simulink model "DualActiveBridgeConverter"  (R2026a)
settings: Solver=ode23t  StopTime=0.010  MaxStep=1e-5  AbsTol=1e-3
PreLoadFcn:
  | DABDefaultInputParameters;
model workspace (MAT data in the model file):
  ConverterKey : string (value not decoded)
undefined symbols (not defined in the file): DABController, DABDesign
libraries: ee_lib x45, nesl_utility x38, fl_lib x19, ConverterLibrary x1, simulink_extras x1
(part 3 of 5)

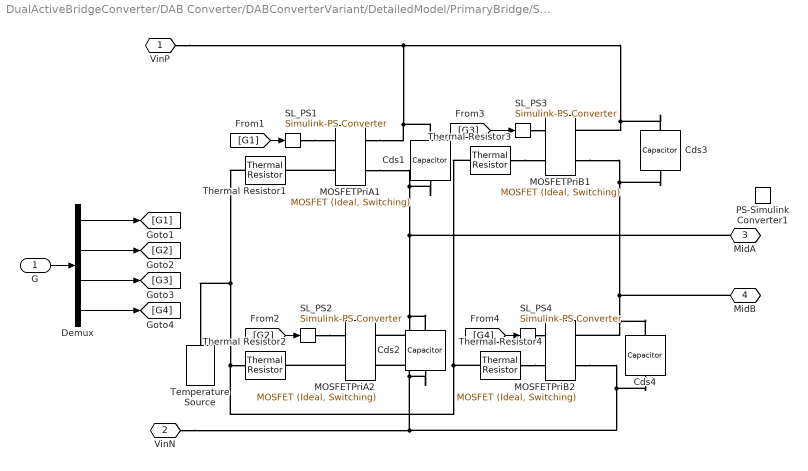
== system DualActiveBridgeConverter/DAB Converter/DABConverterVariant/DetailedModel/PrimaryBridge/SwitchingMOSFETwithThermal ==
  G : Inport
  Cds{1..4} (4 alike) : ee_lib/Passive/Capacitor  cap_option=ee.enum.passive.capacitor.capOption.const  c=CossPri_SI F  Cvec=[1e-05, 1e-06] F  Vvec=[0, 10] V  CV_table_symmetry=ee.enum.passive.capacitor.tableSymmetry.yes  f_vec=[1, 10] kHz  DFext_vec=[.8, 1.2]  enable_C_tol=ee.enum.toleranceApplication.none  averaging_period=0 s  C_tol=5  tol_distribution=ee.enum.toleranceDistribution.uniform  nSigma=4  r=0.05 Ohm  g=1e-5 1/Ohm  enable_operating_limits=ee.enum.enable.no  operating_limit_action=ee.enum.passive.reportOpLim.warn  max_working_voltage_range=[-25, 25] V  power_rating=1 W  maxTemperature=85 degC  thermalEnable=false  thermalMass=1 J/K  i_specify=off  i_priority=None  i=0 A  i_nominal_specify=off  i_nominal_value=1  i_nominal_unit=A  v_specify=off  v_priority=None  v=0 V  v_nominal_specify=off  v_nominal_value=1  v_nominal_unit=V  vc_specify=on  vc_priority=None  vc=0 V  vc_nominal_specify=off  vc_nominal_value=1  vc_nominal_unit=V  T_specify=off  T_priority=None  T=298.15 K  T_nominal_specify=off  T_nominal_value=1  T_nominal_unit=K
  Demux : Demux
  MOSFETPriA1 : ee_lib/Semiconductors & Converters/MOSFET (Ideal, Switching)  PartSpecification="{\"CollectionId\":\"MW.SimscapeElectrical\",\"CollectionVersion\":\"1.0.0\",\"DatasetId\":\"Wolfspeed|C2M0080120D|simscape.electrical.mosfetIdealSwitching\",\"DisplayName\":\"Wolfspeed:C2M0080120D\"}"  port_option=ee.enum.controlport.ps  Rds=0.08 % Datasheet derived Ohm  Goff=8.33333333333333e-10 % Datasheet derived S  Vth=2.9 % Datasheet derived V  diode_param=ee.enum.semiconductors.protectionDiode.nodynamics  diode_Vf=2.47 % Datasheet derived V  diode_Ron=0.031 % Wolfspeed XML derived Ohm  diode_Goff=1e-05 % Library default S  diode_C=50e-9 % Parameter not set F  diode_iRM=-235 % Parameter not set A  diode_iF=300 % Parameter not set A  diode_idot=-50 % Parameter not set A/us  diode_trr_param=ee.enum.converters.diodeReverseParam.trr_factor  diode_trr_factor=3 % Parameter not set  diode_trr=15 % Parameter not set us  diode_Qrr=1500 % Parameter not set s*uA  ids_specify=off  ids_priority=None  ids=0 A  ids_nominal_specify=off  ids_nominal_value=1  ids_nominal_unit=A  vds_specify=off  vds_priority=None  vds=0 V  vds_nominal_specify=off  vds_nominal_value=1  vds_nominal_unit=V  vgs_specify=off  vgs_priority=None  vgs=0 V  vgs_nominal_specify=off  vgs_nominal_value=1  vgs_nominal_unit=V  thermal_loss_option=ee.enum.converters.thermalLossOption.tabulated2d  Von_data=[-3.8 -2.8 -1.8 -1.25 -0.68 -0.35 -0.215 -0.07 0 0.05406 0.21 0.38 0.78 1.6 2.42 3.47 4.66 4.96;-5 -3.49 -2.12 -1.43 -0.746 -0.376 -0.225 -0.074 0 0.075 0.153 0.386 0.785 1.66 2.65 3.85 5.34 5.7;-5.3 -4.56 -3.66 -2.61 -1.344 -0.68 -0.41 -0.15 0 0.152 0.31 0.74 1.44 3 4.97 7.58 11.32 12.44;-6.36 -5.472 -4.392 -3.132 -1.6128 -0.816 -0.492 -0.18 0 0.1824 0.372 0.888 1.728 3.6 5.964 9.096 13.584 14.928] % Wolfspeed XML derived V  Tj=[-55 25 150 900] % Wolfspeed XML derived degC  Iout_data=[-70 -50 -30 -20 -10 -5 -3 -1 0 1 3 5 10 20 30 40 50 52] % Wolfspeed XML derived A  tabulateWithVds=true  Eon_data=[0 0.000124976993 0.00019839481 0.000290262596 0.000394695025 0.000523309904 0.000664552409 0.000828222079 0.001003319539;0 0.000124640962 0.0001962155 0.000286135235 0.000385392686 0.000510053121 0.00064771759 0.000807241087 0.000977902879;0 0.000123102531 0.000190031631 0.000279362347 0.000372104061 0.000492143088 0.0006249736 0.000778895581 0.000943564745;0 0.000122189781 0.000189721879 0.000280387095 0.000371182205 0.000491705578 0.000624418005 0.00077820315 0.000942725925;0 9.7751825e-05 0.000151777503 0.000224309676 0.000296945764 0.000393364462 0.000499534404 0.00062256252 0.00075418074] % Wolfspeed XML derived J  Eoff_data=[0 2.7034922e-05 2.6405907e-05 2.8222037e-05 4.6178646e-05 7.2338984e-05 0.000103764515 0.000172183844 0.000226354181;0 2.7736404e-05 2.7071047e-05 2.901408e-05 4.8053099e-05 7.444232e-05 0.000106781584 0.000177190281 0.000232935681;0 2.8327181e-05 2.7741775e-05 2.9983555e-05 5.0035781e-05 7.7828104e-05 0.000111638221 0.000185249245 0.000243530056;0 2.8334748e-05 2.8341663e-05 3.154355e-05 5.2631616e-05 8.0707822e-05 0.000115768947 0.000192103652 0.000252540911;0 3.4001697e-05 3.4009995e-05 3.785226e-05 6.3157939e-05 9.6849386e-05 0.000138922737 0.000230524383 0.000303049093] % Wolfspeed XML derived J  Eon_data_3D=reshape([0;0;0;0;0;0;0;0;0;0;0;0;0;0;0;0;0;0;0;0;0;0;0;0;0;0;0;0;0;0;0;0;0;0;0;0;0;0;0;0;0;0;0;0;0;0;0;0;0;0;0;0;0;0;0;0;0;0;0;0;0;0;0;0;0;0;0;0;0;0;0;0;0;0;0;0;0;0;0;0;0;0;0;0;0;0;0;0;0;0;0;0;0;0;0;8.0560812e-05;8.0344205e-05;7.9352525e-05;7.8764161e-05;6.3011329e-05;0.00013000148;0.000128573451;0.000124521369;0.000124318399;9.9454719e-05;0.000196389357;0.000193596818;0.000189014336;0.000189707672;0.000151766137;0.000270014001;0.000263650198;0.000254559344;0.000253928694;0.000203142956;0.000365443107;0.000356185495;0.000343678379;0.000343372852;0.000274698281;0.000469433942;0.000457541975;0.000441475822;0.000441083354;0.000352866683;0.00058790882;0.00057301558;0.000552894681;0.000552403162;0.00044192253;0.000724469353;0.000706116684;0.000681322066;0.000680716377;0.000544573101;0;0;0;0;0;0.000124976993;0.000124640962;0.000123102531;0.000122189781;9.7751825e-05;0.00019839481;0.0001962155;0.000190031631;0.000189721879;0.000151777503;0.000290262596;0.000286135235;0.000279362347;0.000280387095;0.000224309676;0.000394695025;0.000385392686;0.000372104061;0.000371182205;0.000296945764;0.000523309904;0.000510053121;0.000492143088;0.000491705578;0.000393364462;0.000664552409;0.00064771759;0.0006249736;0.000624418005;0.000499534404;0.000828222079;0.000807241087;0.000778895581;0.00077820315;0.00062256252;0.001003319539;0.000977902879;0.000943564745;0.000942725925;0.00075418074],[5 9 4]) % Wolfspeed XML derived J  Eoff_data_3D=reshape([0;0;0;0;0;0;0;0;0;0;0;0;0;0;0;0;0;0;0;0;0;0;0;0;0;0;0;0;0;0;0;0;0;0;0;0;0;0;0;0;0;0;0;0;0;0;0;0;0;0;0;0;0;0;0;0;0;0;0;0;0;0;0;0;0;0;0;0;0;0;0;0;0;0;0;0;0;0;0;0;0;0;0;0;0;0;0;0;0;0;0;0;0;0;0;1.7265625e-05;1.7713621e-05;1.8090916e-05;1.8095748e-05;2.1714898e-05;1.5629082e-05;1.6022764e-05;1.6419753e-05;1.6774814e-05;2.0129777e-05;1.8332459e-05;1.8846954e-05;1.9476705e-05;2.0490046e-05;2.4588055e-05;3.1702259e-05;3.2989096e-05;3.4350234e-05;3.6132309e-05;4.3358771e-05;5.1589831e-05;5.3089863e-05;5.5504495e-05;5.7558217e-05;6.906986e-05;8.8425554e-05;9.0996626e-05;9.5135332e-05;9.8655434e-05;0.000118386521;0.000127762888;0.000131477737;0.000137457604;0.000142543673;0.000171052407;0.000173370104;0.000178411033;0.000186525519;0.00019342715;0.000232112579;0;0;0;0;0;2.7034922e-05;2.7736404e-05;2.8327181e-05;2.8334748e-05;3.4001697e-05;2.6405907e-05;2.7071047e-05;2.7741775e-05;2.8341663e-05;3.4009995e-05;2.8222037e-05;2.901408e-05;2.9983555e-05;3.154355e-05;3.785226e-05;4.6178646e-05;4.8053099e-05;5.0035781e-05;5.2631616e-05;6.3157939e-05;7.2338984e-05;7.444232e-05;7.7828104e-05;8.0707822e-05;9.6849386e-05;0.000103764515;0.000106781584;0.000111638221;0.000115768947;0.000138922737;0.000172183844;0.000177190281;0.000185249245;0.000192103652;0.000230524383;0.000226354181;0.000232935681;0.000243530056;0.000252540911;0.000303049093],[5 9 4]) % Wolfspeed XML derived J  Tj_loss=[25 75 125 150 900] % Wolfspeed XML derived degC  Iout_data_loss=[0 4.08 8.4 12.48 16.32 20.4 24.24 27.84 31.68] % Wolfspeed XML derived A  Vds_loss=[-10 0 600 800] % Wolfspeed XML derived V  Eon_scalar=22.86e-3 % Parameter not set J  Eoff_scalar=17.14e-3 % Parameter not set J  Voff=300 % Parameter not set V  Iout_scalar=600 % Parameter not set A  useCurrentFromPreviousCycle=false  useVoltageFromPreviousCycle=false  diodeModelType=ee.enum.converters.diodeModelType.tabulated  diodeTableType=ee.enum.diode.tableType.VfMat  diode_ReverseIVType=ee.enum.diode.diodeReverseIV.constant  diode_IfMat=[.07, .12, .19, 1.75, 4.24, 7.32, 11.2; .16, .3, .72, 2.14, 4.02, 6.35, 9.12] % Parameter not set A  diode_VfMat=[0 3.27 3.6 3.85 4.4 4.95 5.7 6.25 7 7.62;0 2.8 3.16 3.4 3.8 4.25 4.85 5.3 6 6.6;0 2.52 2.76 2.97 3.36 3.78 4.35 4.8 5.5 6.1;0 2.016 2.208 2.376 2.688 3.024 3.48 3.84 4.4 4.88] % Wolfspeed XML derived V  diode_TjVec=[-55 25 150 900] % Wolfspeed XML derived degC  diode_VfVec=[.5, .7, .9, 1.3, 1.7, 2.1, 2.5] % Parameter not set V  diode_IfVec=[0 0.3 1 2 5 10 20 30 50 70] % Wolfspeed XML derived A  diode_IrMat=[1e-06, 2e-06, 5e-06, 1e-05, 2.5e-05, 5e-05, .0001; 2e-06, 5e-06, 1e-05, 4e-05, 8e-05, .0002, .0005] % Parameter not set A  diode_VrMat=[10, 100, 200, 250, 300, 325, 350; 10, 70, 160, 220, 270, 300, 320] % Parameter not set V  diode_VrVec=[10, 20, 40, 50, 70, 80, 100] % Parameter not set V  diode_IrVec=[1e-06, 2e-06, 5e-06, 1e-05, 2e-05, 5e-05, .0001] % Parameter not set A  diode_Vr=-600 % Parameter not set V  diode_Ls=150 % Parameter not set nH  diode_Erec=0.03 % Parameter not set J  diode_rec_loss_model=ee.enum.diode.reverseRecoveryModelTabulateUpTo3D.fixed  diode_ErecVal=0 % Parameter not set J  diode_scaleWithIandV=false  diode_ErecMat=[0 0;0 0] % Wolfspeed XML derived J  diodeErecMat3D=zeros(2, 3, 2) % Parameter not set J  diode_TjrecVec=[25 35] % Wolfspeed XML derived degC  diode_IfrecVec=[0 10] % Wolfspeed XML derived A  diodeVrecVec=[0, 100] % Parameter not set V  diode_IrecVal=10 % Parameter not set A  diode_VrecVal=10 % Wolfspeed XML derived V  diode_tFilter=1 / 1000 / 100 % Parameter not set s  separateThermalPortForDiode=false  thermal_network_parameterization=ee.enum.thermalNetworkTopology.external  Rth=[.03, .2] % Parameter not set K/W  Rth_Cauer=[0.00956 0.242 0.167 0.228] % Wolfspeed XML derived K/W  Rth_Foster=[.08, .14, .22, .16] % Parameter not set K/W  thermal_mass_parameterization=ee.enum.thermalNetwork.thermalmass  thermal_mass=[3, 25] % Parameter not set J/K  thermal_mass_Cauer=[0.00156 0.00604 0.0619 0.358] % Wolfspeed XML derived J/K  thermal_mass_Foster=[.001, .005, .05, .5] % Parameter not set J/K  thermal_time_constant=[.1, 5] % Parameter not set s  thermal_time_constant_Cauer=[.1, 1, 5] % Parameter not set s  thermal_time_constant_Foster=[7e-05, .0007, .01, .08] % Parameter not set s  thermal_mass_initial_temperatures=[25, 25] % Parameter not set degC  thermal_mass_initial_temperatures_Cauer=[25 25 25 25] % Wolfspeed XML derived degC  junction_thermal_mass=0.1 % Parameter not set J/K  Tvec_initial_Foster=[25, 25, 25, 25] % Parameter not set degC  RthDiode=[.03, .2] % Parameter not set K/W  RthCauerDiode=[0.00956 0.242 0.167 0.228] % Wolfspeed XML derived K/W  RthFosterDiode=[.03, .2] % Parameter not set K/W  thermalMassDiode=[3, 25] % Parameter not set J/K  thermalMassCauerDiode=[0.00156 0.00604 0.0619 0.358] % Wolfspeed XML derived J/K  thermalMassFosterDiode=[33, 50] % Parameter not set J/K  thermalTauDiode=[.1, 5] % Parameter not set s  thermalTauCauerDiode=[.1, 1, 5] % Parameter not set s  thermalTauFosterDiode=[1, 10] % Parameter not set s  thermalMassInitTempDiode=[25, 25] % Parameter not set degC  thermalMassInitTempCauerDiode=[25 25 25 25] % Wolfspeed XML derived degC  junctionthermalMassDiode=0.1 % Parameter not set J/K  TVecInitialFosterDiode=[25, 25, 25, 25] % Parameter not set degC  no_thermal_network=0 % Parameter not set  mosfet_junction_temperature_specify=on  mosfet_junction_temperature_priority=High  mosfet_junction_temperature=simTempPri_K K  mosfet_junction_temperature_nominal_specify=off  mosfet_junction_temperature_nominal_value=1  mosfet_junction_temperature_nominal_unit=degC  diode_junction_temperature_specify=off  diode_junction_temperature_priority=None  diode_junction_temperature=simTempPri_K K  diode_junction_temperature_nominal_specify=off  diode_junction_temperature_nominal_value=1  diode_junction_temperature_nominal_unit=degC  Qj_specify=off  Qj_priority=None  Qj=0 W  Qj_nominal_specify=off  Qj_nominal_value=1  Qj_nominal_unit=W  accumulatedSwitchingLosses_specify=off  accumulatedSwitchingLosses_priority=None  accumulatedSwitchingLosses=0 J
      settings: AttributesFormatString=Wolfspeed:C2M0080120D
  MOSFETPriA2 : ee_lib/Semiconductors & Converters/MOSFET (Ideal, Switching)  PartSpecification="{\"CollectionId\":\"MW.SimscapeElectrical\",\"CollectionVersion\":\"1.0.0\",\"DatasetId\":\"Wolfspeed|C2M0080120D|simscape.electrical.mosfetIdealSwitching\",\"DisplayName\":\"Wolfspeed:C2M0080120D\"}"  port_option=ee.enum.controlport.ps  Rds=0.08 % Datasheet derived Ohm  Goff=8.33333333333333e-10 % Datasheet derived S  Vth=2.9 % Datasheet derived V  diode_param=ee.enum.semiconductors.protectionDiode.nodynamics  diode_Vf=2.47 % Datasheet derived V  diode_Ron=0.031 % Wolfspeed XML derived Ohm  diode_Goff=1e-05 % Library default S  diode_C=50e-9 % Parameter not set F  diode_iRM=-235 % Parameter not set A  diode_iF=300 % Parameter not set A  diode_idot=-50 % Parameter not set A/us  diode_trr_param=ee.enum.converters.diodeReverseParam.trr_factor  diode_trr_factor=3 % Parameter not set  diode_trr=15 % Parameter not set us  diode_Qrr=1500 % Parameter not set s*uA  ids_specify=off  ids_priority=None  ids=0 A  ids_nominal_specify=off  ids_nominal_value=1  ids_nominal_unit=A  vds_specify=off  vds_priority=None  vds=0 V  vds_nominal_specify=off  vds_nominal_value=1  vds_nominal_unit=V  vgs_specify=off  vgs_priority=None  vgs=0 V  vgs_nominal_specify=off  vgs_nominal_value=1  vgs_nominal_unit=V  thermal_loss_option=ee.enum.converters.thermalLossOption.tabulated2d  Von_data=[-3.8 -2.8 -1.8 -1.25 -0.68 -0.35 -0.215 -0.07 0 0.05406 0.21 0.38 0.78 1.6 2.42 3.47 4.66 4.96;-5 -3.49 -2.12 -1.43 -0.746 -0.376 -0.225 -0.074 0 0.075 0.153 0.386 0.785 1.66 2.65 3.85 5.34 5.7;-5.3 -4.56 -3.66 -2.61 -1.344 -0.68 -0.41 -0.15 0 0.152 0.31 0.74 1.44 3 4.97 7.58 11.32 12.44;-6.36 -5.472 -4.392 -3.132 -1.6128 -0.816 -0.492 -0.18 0 0.1824 0.372 0.888 1.728 3.6 5.964 9.096 13.584 14.928] % Wolfspeed XML derived V  Tj=[-55 25 150 900] % Wolfspeed XML derived degC  Iout_data=[-70 -50 -30 -20 -10 -5 -3 -1 0 1 3 5 10 20 30 40 50 52] % Wolfspeed XML derived A  tabulateWithVds=true  Eon_data=[0 0.000124976993 0.00019839481 0.000290262596 0.000394695025 0.000523309904 0.000664552409 0.000828222079 0.001003319539;0 0.000124640962 0.0001962155 0.000286135235 0.000385392686 0.000510053121 0.00064771759 0.000807241087 0.000977902879;0 0.000123102531 0.000190031631 0.000279362347 0.000372104061 0.000492143088 0.0006249736 0.000778895581 0.000943564745;0 0.000122189781 0.000189721879 0.000280387095 0.000371182205 0.000491705578 0.000624418005 0.00077820315 0.000942725925;0 9.7751825e-05 0.000151777503 0.000224309676 0.000296945764 0.000393364462 0.000499534404 0.00062256252 0.00075418074] % Wolfspeed XML derived J  Eoff_data=[0 2.7034922e-05 2.6405907e-05 2.8222037e-05 4.6178646e-05 7.2338984e-05 0.000103764515 0.000172183844 0.000226354181;0 2.7736404e-05 2.7071047e-05 2.901408e-05 4.8053099e-05 7.444232e-05 0.000106781584 0.000177190281 0.000232935681;0 2.8327181e-05 2.7741775e-05 2.9983555e-05 5.0035781e-05 7.7828104e-05 0.000111638221 0.000185249245 0.000243530056;0 2.8334748e-05 2.8341663e-05 3.154355e-05 5.2631616e-05 8.0707822e-05 0.000115768947 0.000192103652 0.000252540911;0 3.4001697e-05 3.4009995e-05 3.785226e-05 6.3157939e-05 9.6849386e-05 0.000138922737 0.000230524383 0.000303049093] % Wolfspeed XML derived J  Eon_data_3D=reshape([0;0;0;0;0;0;0;0;0;0;0;0;0;0;0;0;0;0;0;0;0;0;0;0;0;0;0;0;0;0;0;0;0;0;0;0;0;0;0;0;0;0;0;0;0;0;0;0;0;0;0;0;0;0;0;0;0;0;0;0;0;0;0;0;0;0;0;0;0;0;0;0;0;0;0;0;0;0;0;0;0;0;0;0;0;0;0;0;0;0;0;0;0;0;0;8.0560812e-05;8.0344205e-05;7.9352525e-05;7.8764161e-05;6.3011329e-05;0.00013000148;0.000128573451;0.000124521369;0.000124318399;9.9454719e-05;0.000196389357;0.000193596818;0.000189014336;0.000189707672;0.000151766137;0.000270014001;0.000263650198;0.000254559344;0.000253928694;0.000203142956;0.000365443107;0.000356185495;0.000343678379;0.000343372852;0.000274698281;0.000469433942;0.000457541975;0.000441475822;0.000441083354;0.000352866683;0.00058790882;0.00057301558;0.000552894681;0.000552403162;0.00044192253;0.000724469353;0.000706116684;0.000681322066;0.000680716377;0.000544573101;0;0;0;0;0;0.000124976993;0.000124640962;0.000123102531;0.000122189781;9.7751825e-05;0.00019839481;0.0001962155;0.000190031631;0.000189721879;0.000151777503;0.000290262596;0.000286135235;0.000279362347;0.000280387095;0.000224309676;0.000394695025;0.000385392686;0.000372104061;0.000371182205;0.000296945764;0.000523309904;0.000510053121;0.000492143088;0.000491705578;0.000393364462;0.000664552409;0.00064771759;0.0006249736;0.000624418005;0.000499534404;0.000828222079;0.000807241087;0.000778895581;0.00077820315;0.00062256252;0.001003319539;0.000977902879;0.000943564745;0.000942725925;0.00075418074],[5 9 4]) % Wolfspeed XML derived J  Eoff_data_3D=reshape([0;0;0;0;0;0;0;0;0;0;0;0;0;0;0;0;0;0;0;0;0;0;0;0;0;0;0;0;0;0;0;0;0;0;0;0;0;0;0;0;0;0;0;0;0;0;0;0;0;0;0;0;0;0;0;0;0;0;0;0;0;0;0;0;0;0;0;0;0;0;0;0;0;0;0;0;0;0;0;0;0;0;0;0;0;0;0;0;0;0;0;0;0;0;0;1.7265625e-05;1.7713621e-05;1.8090916e-05;1.8095748e-05;2.1714898e-05;1.5629082e-05;1.6022764e-05;1.6419753e-05;1.6774814e-05;2.0129777e-05;1.8332459e-05;1.8846954e-05;1.9476705e-05;2.0490046e-05;2.4588055e-05;3.1702259e-05;3.2989096e-05;3.4350234e-05;3.6132309e-05;4.3358771e-05;5.1589831e-05;5.3089863e-05;5.5504495e-05;5.7558217e-05;6.906986e-05;8.8425554e-05;9.0996626e-05;9.5135332e-05;9.8655434e-05;0.000118386521;0.000127762888;0.000131477737;0.000137457604;0.000142543673;0.000171052407;0.000173370104;0.000178411033;0.000186525519;0.00019342715;0.000232112579;0;0;0;0;0;2.7034922e-05;2.7736404e-05;2.8327181e-05;2.8334748e-05;3.4001697e-05;2.6405907e-05;2.7071047e-05;2.7741775e-05;2.8341663e-05;3.4009995e-05;2.8222037e-05;2.901408e-05;2.9983555e-05;3.154355e-05;3.785226e-05;4.6178646e-05;4.8053099e-05;5.0035781e-05;5.2631616e-05;6.3157939e-05;7.2338984e-05;7.444232e-05;7.7828104e-05;8.0707822e-05;9.6849386e-05;0.000103764515;0.000106781584;0.000111638221;0.000115768947;0.000138922737;0.000172183844;0.000177190281;0.000185249245;0.000192103652;0.000230524383;0.000226354181;0.000232935681;0.000243530056;0.000252540911;0.000303049093],[5 9 4]) % Wolfspeed XML derived J  Tj_loss=[25 75 125 150 900] % Wolfspeed XML derived degC  Iout_data_loss=[0 4.08 8.4 12.48 16.32 20.4 24.24 27.84 31.68] % Wolfspeed XML derived A  Vds_loss=[-10 0 600 800] % Wolfspeed XML derived V  Eon_scalar=22.86e-3 % Parameter not set J  Eoff_scalar=17.14e-3 % Parameter not set J  Voff=300 % Parameter not set V  Iout_scalar=600 % Parameter not set A  useCurrentFromPreviousCycle=false  useVoltageFromPreviousCycle=false  diodeModelType=ee.enum.converters.diodeModelType.tabulated  diodeTableType=ee.enum.diode.tableType.VfMat  diode_ReverseIVType=ee.enum.diode.diodeReverseIV.constant  diode_IfMat=[.07, .12, .19, 1.75, 4.24, 7.32, 11.2; .16, .3, .72, 2.14, 4.02, 6.35, 9.12] % Parameter not set A  diode_VfMat=[0 3.27 3.6 3.85 4.4 4.95 5.7 6.25 7 7.62;0 2.8 3.16 3.4 3.8 4.25 4.85 5.3 6 6.6;0 2.52 2.76 2.97 3.36 3.78 4.35 4.8 5.5 6.1;0 2.016 2.208 2.376 2.688 3.024 3.48 3.84 4.4 4.88] % Wolfspeed XML derived V  diode_TjVec=[-55 25 150 900] % Wolfspeed XML derived degC  diode_VfVec=[.5, .7, .9, 1.3, 1.7, 2.1, 2.5] % Parameter not set V  diode_IfVec=[0 0.3 1 2 5 10 20 30 50 70] % Wolfspeed XML derived A  diode_IrMat=[1e-06, 2e-06, 5e-06, 1e-05, 2.5e-05, 5e-05, .0001; 2e-06, 5e-06, 1e-05, 4e-05, 8e-05, .0002, .0005] % Parameter not set A  diode_VrMat=[10, 100, 200, 250, 300, 325, 350; 10, 70, 160, 220, 270, 300, 320] % Parameter not set V  diode_VrVec=[10, 20, 40, 50, 70, 80, 100] % Parameter not set V  diode_IrVec=[1e-06, 2e-06, 5e-06, 1e-05, 2e-05, 5e-05, .0001] % Parameter not set A  diode_Vr=-600 % Parameter not set V  diode_Ls=150 % Parameter not set nH  diode_Erec=0.03 % Parameter not set J  diode_rec_loss_model=ee.enum.diode.reverseRecoveryModelTabulateUpTo3D.fixed  diode_ErecVal=0 % Parameter not set J  diode_scaleWithIandV=false  diode_ErecMat=[0 0;0 0] % Wolfspeed XML derived J  diodeErecMat3D=zeros(2, 3, 2) % Parameter not set J  diode_TjrecVec=[25 35] % Wolfspeed XML derived degC  diode_IfrecVec=[0 10] % Wolfspeed XML derived A  diodeVrecVec=[0, 100] % Parameter not set V  diode_IrecVal=10 % Parameter not set A  diode_VrecVal=10 % Wolfspeed XML derived V  diode_tFilter=1 / 1000 / 100 % Parameter not set s  separateThermalPortForDiode=false  thermal_network_parameterization=ee.enum.thermalNetworkTopology.external  Rth=[.03, .2] % Parameter not set K/W  Rth_Cauer=[0.00956 0.242 0.167 0.228] % Wolfspeed XML derived K/W  Rth_Foster=[.08, .14, .22, .16] % Parameter not set K/W  thermal_mass_parameterization=ee.enum.thermalNetwork.thermalmass  thermal_mass=[3, 25] % Parameter not set J/K  thermal_mass_Cauer=[0.00156 0.00604 0.0619 0.358] % Wolfspeed XML derived J/K  thermal_mass_Foster=[.001, .005, .05, .5] % Parameter not set J/K  thermal_time_constant=[.1, 5] % Parameter not set s  thermal_time_constant_Cauer=[.1, 1, 5] % Parameter not set s  thermal_time_constant_Foster=[7e-05, .0007, .01, .08] % Parameter not set s  thermal_mass_initial_temperatures=[25, 25] % Parameter not set degC  thermal_mass_initial_temperatures_Cauer=[25 25 25 25] % Wolfspeed XML derived degC  junction_thermal_mass=0.1 % Parameter not set J/K  Tvec_initial_Foster=[25, 25, 25, 25] % Parameter not set degC  RthDiode=[.03, .2] % Parameter not set K/W  RthCauerDiode=[0.00956 0.242 0.167 0.228] % Wolfspeed XML derived K/W  RthFosterDiode=[.03, .2] % Parameter not set K/W  thermalMassDiode=[3, 25] % Parameter not set J/K  thermalMassCauerDiode=[0.00156 0.00604 0.0619 0.358] % Wolfspeed XML derived J/K  thermalMassFosterDiode=[33, 50] % Parameter not set J/K  thermalTauDiode=[.1, 5] % Parameter not set s  thermalTauCauerDiode=[.1, 1, 5] % Parameter not set s  thermalTauFosterDiode=[1, 10] % Parameter not set s  thermalMassInitTempDiode=[25, 25] % Parameter not set degC  thermalMassInitTempCauerDiode=[25 25 25 25] % Wolfspeed XML derived degC  junctionthermalMassDiode=0.1 % Parameter not set J/K  TVecInitialFosterDiode=[25, 25, 25, 25] % Parameter not set degC  no_thermal_network=0 % Parameter not set  mosfet_junction_temperature_specify=on  mosfet_junction_temperature_priority=High  mosfet_junction_temperature=simTempPri_K K  mosfet_junction_temperature_nominal_specify=off  mosfet_junction_temperature_nominal_value=1  mosfet_junction_temperature_nominal_unit=degC  diode_junction_temperature_specify=off  diode_junction_temperature_priority=None  diode_junction_temperature=simTempPri_K K  diode_junction_temperature_nominal_specify=off  diode_junction_temperature_nominal_value=1  diode_junction_temperature_nominal_unit=degC  Qj_specify=off  Qj_priority=None  Qj=0 W  Qj_nominal_specify=off  Qj_nominal_value=1  Qj_nominal_unit=W  accumulatedSwitchingLosses_specify=off  accumulatedSwitchingLosses_priority=None  accumulatedSwitchingLosses=0 J
      settings: AttributesFormatString=Wolfspeed:C2M0080120D
  MOSFETPriB1 : ee_lib/Semiconductors & Converters/MOSFET (Ideal, Switching)  PartSpecification="{\"CollectionId\":\"MW.SimscapeElectrical\",\"CollectionVersion\":\"1.0.0\",\"DatasetId\":\"Wolfspeed|C2M0080120D|simscape.electrical.mosfetIdealSwitching\",\"DisplayName\":\"Wolfspeed:C2M0080120D\"}"  port_option=ee.enum.controlport.ps  Rds=0.08 % Datasheet derived Ohm  Goff=8.33333333333333e-10 % Datasheet derived S  Vth=2.9 % Datasheet derived V  diode_param=ee.enum.semiconductors.protectionDiode.nodynamics  diode_Vf=2.47 % Datasheet derived V  diode_Ron=0.031 % Wolfspeed XML derived Ohm  diode_Goff=1e-05 % Library default S  diode_C=50e-9 % Parameter not set F  diode_iRM=-235 % Parameter not set A  diode_iF=300 % Parameter not set A  diode_idot=-50 % Parameter not set A/us  diode_trr_param=ee.enum.converters.diodeReverseParam.trr_factor  diode_trr_factor=3 % Parameter not set  diode_trr=15 % Parameter not set us  diode_Qrr=1500 % Parameter not set s*uA  ids_specify=off  ids_priority=None  ids=0 A  ids_nominal_specify=off  ids_nominal_value=1  ids_nominal_unit=A  vds_specify=off  vds_priority=None  vds=0 V  vds_nominal_specify=off  vds_nominal_value=1  vds_nominal_unit=V  vgs_specify=off  vgs_priority=None  vgs=0 V  vgs_nominal_specify=off  vgs_nominal_value=1  vgs_nominal_unit=V  thermal_loss_option=ee.enum.converters.thermalLossOption.tabulated2d  Von_data=[-3.8 -2.8 -1.8 -1.25 -0.68 -0.35 -0.215 -0.07 0 0.05406 0.21 0.38 0.78 1.6 2.42 3.47 4.66 4.96;-5 -3.49 -2.12 -1.43 -0.746 -0.376 -0.225 -0.074 0 0.075 0.153 0.386 0.785 1.66 2.65 3.85 5.34 5.7;-5.3 -4.56 -3.66 -2.61 -1.344 -0.68 -0.41 -0.15 0 0.152 0.31 0.74 1.44 3 4.97 7.58 11.32 12.44;-6.36 -5.472 -4.392 -3.132 -1.6128 -0.816 -0.492 -0.18 0 0.1824 0.372 0.888 1.728 3.6 5.964 9.096 13.584 14.928] % Wolfspeed XML derived V  Tj=[-55 25 150 900] % Wolfspeed XML derived degC  Iout_data=[-70 -50 -30 -20 -10 -5 -3 -1 0 1 3 5 10 20 30 40 50 52] % Wolfspeed XML derived A  tabulateWithVds=true  Eon_data=[0 0.000124976993 0.00019839481 0.000290262596 0.000394695025 0.000523309904 0.000664552409 0.000828222079 0.001003319539;0 0.000124640962 0.0001962155 0.000286135235 0.000385392686 0.000510053121 0.00064771759 0.000807241087 0.000977902879;0 0.000123102531 0.000190031631 0.000279362347 0.000372104061 0.000492143088 0.0006249736 0.000778895581 0.000943564745;0 0.000122189781 0.000189721879 0.000280387095 0.000371182205 0.000491705578 0.000624418005 0.00077820315 0.000942725925;0 9.7751825e-05 0.000151777503 0.000224309676 0.000296945764 0.000393364462 0.000499534404 0.00062256252 0.00075418074] % Wolfspeed XML derived J  Eoff_data=[0 2.7034922e-05 2.6405907e-05 2.8222037e-05 4.6178646e-05 7.2338984e-05 0.000103764515 0.000172183844 0.000226354181;0 2.7736404e-05 2.7071047e-05 2.901408e-05 4.8053099e-05 7.444232e-05 0.000106781584 0.000177190281 0.000232935681;0 2.8327181e-05 2.7741775e-05 2.9983555e-05 5.0035781e-05 7.7828104e-05 0.000111638221 0.000185249245 0.000243530056;0 2.8334748e-05 2.8341663e-05 3.154355e-05 5.2631616e-05 8.0707822e-05 0.000115768947 0.000192103652 0.000252540911;0 3.4001697e-05 3.4009995e-05 3.785226e-05 6.3157939e-05 9.6849386e-05 0.000138922737 0.000230524383 0.000303049093] % Wolfspeed XML derived J  Eon_data_3D=reshape([0;0;0;0;0;0;0;0;0;0;0;0;0;0;0;0;0;0;0;0;0;0;0;0;0;0;0;0;0;0;0;0;0;0;0;0;0;0;0;0;0;0;0;0;0;0;0;0;0;0;0;0;0;0;0;0;0;0;0;0;0;0;0;0;0;0;0;0;0;0;0;0;0;0;0;0;0;0;0;0;0;0;0;0;0;0;0;0;0;0;0;0;0;0;0;8.0560812e-05;8.0344205e-05;7.9352525e-05;7.8764161e-05;6.3011329e-05;0.00013000148;0.000128573451;0.000124521369;0.000124318399;9.9454719e-05;0.000196389357;0.000193596818;0.000189014336;0.000189707672;0.000151766137;0.000270014001;0.000263650198;0.000254559344;0.000253928694;0.000203142956;0.000365443107;0.000356185495;0.000343678379;0.000343372852;0.000274698281;0.000469433942;0.000457541975;0.000441475822;0.000441083354;0.000352866683;0.00058790882;0.00057301558;0.000552894681;0.000552403162;0.00044192253;0.000724469353;0.000706116684;0.000681322066;0.000680716377;0.000544573101;0;0;0;0;0;0.000124976993;0.000124640962;0.000123102531;0.000122189781;9.7751825e-05;0.00019839481;0.0001962155;0.000190031631;0.000189721879;0.000151777503;0.000290262596;0.000286135235;0.000279362347;0.000280387095;0.000224309676;0.000394695025;0.000385392686;0.000372104061;0.000371182205;0.000296945764;0.000523309904;0.000510053121;0.000492143088;0.000491705578;0.000393364462;0.000664552409;0.00064771759;0.0006249736;0.000624418005;0.000499534404;0.000828222079;0.000807241087;0.000778895581;0.00077820315;0.00062256252;0.001003319539;0.000977902879;0.000943564745;0.000942725925;0.00075418074],[5 9 4]) % Wolfspeed XML derived J  Eoff_data_3D=reshape([0;0;0;0;0;0;0;0;0;0;0;0;0;0;0;0;0;0;0;0;0;0;0;0;0;0;0;0;0;0;0;0;0;0;0;0;0;0;0;0;0;0;0;0;0;0;0;0;0;0;0;0;0;0;0;0;0;0;0;0;0;0;0;0;0;0;0;0;0;0;0;0;0;0;0;0;0;0;0;0;0;0;0;0;0;0;0;0;0;0;0;0;0;0;0;1.7265625e-05;1.7713621e-05;1.8090916e-05;1.8095748e-05;2.1714898e-05;1.5629082e-05;1.6022764e-05;1.6419753e-05;1.6774814e-05;2.0129777e-05;1.8332459e-05;1.8846954e-05;1.9476705e-05;2.0490046e-05;2.4588055e-05;3.1702259e-05;3.2989096e-05;3.4350234e-05;3.6132309e-05;4.3358771e-05;5.1589831e-05;5.3089863e-05;5.5504495e-05;5.7558217e-05;6.906986e-05;8.8425554e-05;9.0996626e-05;9.5135332e-05;9.8655434e-05;0.000118386521;0.000127762888;0.000131477737;0.000137457604;0.000142543673;0.000171052407;0.000173370104;0.000178411033;0.000186525519;0.00019342715;0.000232112579;0;0;0;0;0;2.7034922e-05;2.7736404e-05;2.8327181e-05;2.8334748e-05;3.4001697e-05;2.6405907e-05;2.7071047e-05;2.7741775e-05;2.8341663e-05;3.4009995e-05;2.8222037e-05;2.901408e-05;2.9983555e-05;3.154355e-05;3.785226e-05;4.6178646e-05;4.8053099e-05;5.0035781e-05;5.2631616e-05;6.3157939e-05;7.2338984e-05;7.444232e-05;7.7828104e-05;8.0707822e-05;9.6849386e-05;0.000103764515;0.000106781584;0.000111638221;0.000115768947;0.000138922737;0.000172183844;0.000177190281;0.000185249245;0.000192103652;0.000230524383;0.000226354181;0.000232935681;0.000243530056;0.000252540911;0.000303049093],[5 9 4]) % Wolfspeed XML derived J  Tj_loss=[25 75 125 150 900] % Wolfspeed XML derived degC  Iout_data_loss=[0 4.08 8.4 12.48 16.32 20.4 24.24 27.84 31.68] % Wolfspeed XML derived A  Vds_loss=[-10 0 600 800] % Wolfspeed XML derived V  Eon_scalar=22.86e-3 % Parameter not set J  Eoff_scalar=17.14e-3 % Parameter not set J  Voff=300 % Parameter not set V  Iout_scalar=600 % Parameter not set A  useCurrentFromPreviousCycle=false  useVoltageFromPreviousCycle=false  diodeModelType=ee.enum.converters.diodeModelType.tabulated  diodeTableType=ee.enum.diode.tableType.VfMat  diode_ReverseIVType=ee.enum.diode.diodeReverseIV.constant  diode_IfMat=[.07, .12, .19, 1.75, 4.24, 7.32, 11.2; .16, .3, .72, 2.14, 4.02, 6.35, 9.12] % Parameter not set A  diode_VfMat=[0 3.27 3.6 3.85 4.4 4.95 5.7 6.25 7 7.62;0 2.8 3.16 3.4 3.8 4.25 4.85 5.3 6 6.6;0 2.52 2.76 2.97 3.36 3.78 4.35 4.8 5.5 6.1;0 2.016 2.208 2.376 2.688 3.024 3.48 3.84 4.4 4.88] % Wolfspeed XML derived V  diode_TjVec=[-55 25 150 900] % Wolfspeed XML derived degC  diode_VfVec=[.5, .7, .9, 1.3, 1.7, 2.1, 2.5] % Parameter not set V  diode_IfVec=[0 0.3 1 2 5 10 20 30 50 70] % Wolfspeed XML derived A  diode_IrMat=[1e-06, 2e-06, 5e-06, 1e-05, 2.5e-05, 5e-05, .0001; 2e-06, 5e-06, 1e-05, 4e-05, 8e-05, .0002, .0005] % Parameter not set A  diode_VrMat=[10, 100, 200, 250, 300, 325, 350; 10, 70, 160, 220, 270, 300, 320] % Parameter not set V  diode_VrVec=[10, 20, 40, 50, 70, 80, 100] % Parameter not set V  diode_IrVec=[1e-06, 2e-06, 5e-06, 1e-05, 2e-05, 5e-05, .0001] % Parameter not set A  diode_Vr=-600 % Parameter not set V  diode_Ls=150 % Parameter not set nH  diode_Erec=0.03 % Parameter not set J  diode_rec_loss_model=ee.enum.diode.reverseRecoveryModelTabulateUpTo3D.fixed  diode_ErecVal=0 % Parameter not set J  diode_scaleWithIandV=false  diode_ErecMat=[0 0;0 0] % Wolfspeed XML derived J  diodeErecMat3D=zeros(2, 3, 2) % Parameter not set J  diode_TjrecVec=[25 35] % Wolfspeed XML derived degC  diode_IfrecVec=[0 10] % Wolfspeed XML derived A  diodeVrecVec=[0, 100] % Parameter not set V  diode_IrecVal=10 % Parameter not set A  diode_VrecVal=10 % Wolfspeed XML derived V  diode_tFilter=1 / 1000 / 100 % Parameter not set s  separateThermalPortForDiode=false  thermal_network_parameterization=ee.enum.thermalNetworkTopology.external  Rth=[.03, .2] % Parameter not set K/W  Rth_Cauer=[0.00956 0.242 0.167 0.228] % Wolfspeed XML derived K/W  Rth_Foster=[.08, .14, .22, .16] % Parameter not set K/W  thermal_mass_parameterization=ee.enum.thermalNetwork.thermalmass  thermal_mass=[3, 25] % Parameter not set J/K  thermal_mass_Cauer=[0.00156 0.00604 0.0619 0.358] % Wolfspeed XML derived J/K  thermal_mass_Foster=[.001, .005, .05, .5] % Parameter not set J/K  thermal_time_constant=[.1, 5] % Parameter not set s  thermal_time_constant_Cauer=[.1, 1, 5] % Parameter not set s  thermal_time_constant_Foster=[7e-05, .0007, .01, .08] % Parameter not set s  thermal_mass_initial_temperatures=[25, 25] % Parameter not set degC  thermal_mass_initial_temperatures_Cauer=[25 25 25 25] % Wolfspeed XML derived degC  junction_thermal_mass=0.1 % Parameter not set J/K  Tvec_initial_Foster=[25, 25, 25, 25] % Parameter not set degC  RthDiode=[.03, .2] % Parameter not set K/W  RthCauerDiode=[0.00956 0.242 0.167 0.228] % Wolfspeed XML derived K/W  RthFosterDiode=[.03, .2] % Parameter not set K/W  thermalMassDiode=[3, 25] % Parameter not set J/K  thermalMassCauerDiode=[0.00156 0.00604 0.0619 0.358] % Wolfspeed XML derived J/K  thermalMassFosterDiode=[33, 50] % Parameter not set J/K  thermalTauDiode=[.1, 5] % Parameter not set s  thermalTauCauerDiode=[.1, 1, 5] % Parameter not set s  thermalTauFosterDiode=[1, 10] % Parameter not set s  thermalMassInitTempDiode=[25, 25] % Parameter not set degC  thermalMassInitTempCauerDiode=[25 25 25 25] % Wolfspeed XML derived degC  junctionthermalMassDiode=0.1 % Parameter not set J/K  TVecInitialFosterDiode=[25, 25, 25, 25] % Parameter not set degC  no_thermal_network=0 % Parameter not set  mosfet_junction_temperature_specify=on  mosfet_junction_temperature_priority=High  mosfet_junction_temperature=simTempPri_K K  mosfet_junction_temperature_nominal_specify=off  mosfet_junction_temperature_nominal_value=1  mosfet_junction_temperature_nominal_unit=degC  diode_junction_temperature_specify=off  diode_junction_temperature_priority=None  diode_junction_temperature=simTempPri_K K  diode_junction_temperature_nominal_specify=off  diode_junction_temperature_nominal_value=1  diode_junction_temperature_nominal_unit=degC  Qj_specify=off  Qj_priority=None  Qj=0 W  Qj_nominal_specify=off  Qj_nominal_value=1  Qj_nominal_unit=W  accumulatedSwitchingLosses_specify=off  accumulatedSwitchingLosses_priority=None  accumulatedSwitchingLosses=0 J
      settings: AttributesFormatString=Wolfspeed:C2M0080120D
  MOSFETPriB2 : ee_lib/Semiconductors & Converters/MOSFET (Ideal, Switching)  PartSpecification="{\"CollectionId\":\"MW.SimscapeElectrical\",\"CollectionVersion\":\"1.0.0\",\"DatasetId\":\"Wolfspeed|C2M0080120D|simscape.electrical.mosfetIdealSwitching\",\"DisplayName\":\"Wolfspeed:C2M0080120D\"}"  port_option=ee.enum.controlport.ps  Rds=0.08 % Datasheet derived Ohm  Goff=8.33333333333333e-10 % Datasheet derived S  Vth=2.9 % Datasheet derived V  diode_param=ee.enum.semiconductors.protectionDiode.nodynamics  diode_Vf=2.47 % Datasheet derived V  diode_Ron=0.031 % Wolfspeed XML derived Ohm  diode_Goff=1e-05 % Library default S  diode_C=50e-9 % Parameter not set F  diode_iRM=-235 % Parameter not set A  diode_iF=300 % Parameter not set A  diode_idot=-50 % Parameter not set A/us  diode_trr_param=ee.enum.converters.diodeReverseParam.trr_factor  diode_trr_factor=3 % Parameter not set  diode_trr=15 % Parameter not set us  diode_Qrr=1500 % Parameter not set s*uA  ids_specify=off  ids_priority=None  ids=0 A  ids_nominal_specify=off  ids_nominal_value=1  ids_nominal_unit=A  vds_specify=off  vds_priority=None  vds=0 V  vds_nominal_specify=off  vds_nominal_value=1  vds_nominal_unit=V  vgs_specify=off  vgs_priority=None  vgs=0 V  vgs_nominal_specify=off  vgs_nominal_value=1  vgs_nominal_unit=V  thermal_loss_option=ee.enum.converters.thermalLossOption.tabulated2d  Von_data=[-3.8 -2.8 -1.8 -1.25 -0.68 -0.35 -0.215 -0.07 0 0.05406 0.21 0.38 0.78 1.6 2.42 3.47 4.66 4.96;-5 -3.49 -2.12 -1.43 -0.746 -0.376 -0.225 -0.074 0 0.075 0.153 0.386 0.785 1.66 2.65 3.85 5.34 5.7;-5.3 -4.56 -3.66 -2.61 -1.344 -0.68 -0.41 -0.15 0 0.152 0.31 0.74 1.44 3 4.97 7.58 11.32 12.44;-6.36 -5.472 -4.392 -3.132 -1.6128 -0.816 -0.492 -0.18 0 0.1824 0.372 0.888 1.728 3.6 5.964 9.096 13.584 14.928] % Wolfspeed XML derived V  Tj=[-55 25 150 900] % Wolfspeed XML derived degC  Iout_data=[-70 -50 -30 -20 -10 -5 -3 -1 0 1 3 5 10 20 30 40 50 52] % Wolfspeed XML derived A  tabulateWithVds=true  Eon_data=[0 0.000124976993 0.00019839481 0.000290262596 0.000394695025 0.000523309904 0.000664552409 0.000828222079 0.001003319539;0 0.000124640962 0.0001962155 0.000286135235 0.000385392686 0.000510053121 0.00064771759 0.000807241087 0.000977902879;0 0.000123102531 0.000190031631 0.000279362347 0.000372104061 0.000492143088 0.0006249736 0.000778895581 0.000943564745;0 0.000122189781 0.000189721879 0.000280387095 0.000371182205 0.000491705578 0.000624418005 0.00077820315 0.000942725925;0 9.7751825e-05 0.000151777503 0.000224309676 0.000296945764 0.000393364462 0.000499534404 0.00062256252 0.00075418074] % Wolfspeed XML derived J  Eoff_data=[0 2.7034922e-05 2.6405907e-05 2.8222037e-05 4.6178646e-05 7.2338984e-05 0.000103764515 0.000172183844 0.000226354181;0 2.7736404e-05 2.7071047e-05 2.901408e-05 4.8053099e-05 7.444232e-05 0.000106781584 0.000177190281 0.000232935681;0 2.8327181e-05 2.7741775e-05 2.9983555e-05 5.0035781e-05 7.7828104e-05 0.000111638221 0.000185249245 0.000243530056;0 2.8334748e-05 2.8341663e-05 3.154355e-05 5.2631616e-05 8.0707822e-05 0.000115768947 0.000192103652 0.000252540911;0 3.4001697e-05 3.4009995e-05 3.785226e-05 6.3157939e-05 9.6849386e-05 0.000138922737 0.000230524383 0.000303049093] % Wolfspeed XML derived J  Eon_data_3D=reshape([0;0;0;0;0;0;0;0;0;0;0;0;0;0;0;0;0;0;0;0;0;0;0;0;0;0;0;0;0;0;0;0;0;0;0;0;0;0;0;0;0;0;0;0;0;0;0;0;0;0;0;0;0;0;0;0;0;0;0;0;0;0;0;0;0;0;0;0;0;0;0;0;0;0;0;0;0;0;0;0;0;0;0;0;0;0;0;0;0;0;0;0;0;0;0;8.0560812e-05;8.0344205e-05;7.9352525e-05;7.8764161e-05;6.3011329e-05;0.00013000148;0.000128573451;0.000124521369;0.000124318399;9.9454719e-05;0.000196389357;0.000193596818;0.000189014336;0.000189707672;0.000151766137;0.000270014001;0.000263650198;0.000254559344;0.000253928694;0.000203142956;0.000365443107;0.000356185495;0.000343678379;0.000343372852;0.000274698281;0.000469433942;0.000457541975;0.000441475822;0.000441083354;0.000352866683;0.00058790882;0.00057301558;0.000552894681;0.000552403162;0.00044192253;0.000724469353;0.000706116684;0.000681322066;0.000680716377;0.000544573101;0;0;0;0;0;0.000124976993;0.000124640962;0.000123102531;0.000122189781;9.7751825e-05;0.00019839481;0.0001962155;0.000190031631;0.000189721879;0.000151777503;0.000290262596;0.000286135235;0.000279362347;0.000280387095;0.000224309676;0.000394695025;0.000385392686;0.000372104061;0.000371182205;0.000296945764;0.000523309904;0.000510053121;0.000492143088;0.000491705578;0.000393364462;0.000664552409;0.00064771759;0.0006249736;0.000624418005;0.000499534404;0.000828222079;0.000807241087;0.000778895581;0.00077820315;0.00062256252;0.001003319539;0.000977902879;0.000943564745;0.000942725925;0.00075418074],[5 9 4]) % Wolfspeed XML derived J  Eoff_data_3D=reshape([0;0;0;0;0;0;0;0;0;0;0;0;0;0;0;0;0;0;0;0;0;0;0;0;0;0;0;0;0;0;0;0;0;0;0;0;0;0;0;0;0;0;0;0;0;0;0;0;0;0;0;0;0;0;0;0;0;0;0;0;0;0;0;0;0;0;0;0;0;0;0;0;0;0;0;0;0;0;0;0;0;0;0;0;0;0;0;0;0;0;0;0;0;0;0;1.7265625e-05;1.7713621e-05;1.8090916e-05;1.8095748e-05;2.1714898e-05;1.5629082e-05;1.6022764e-05;1.6419753e-05;1.6774814e-05;2.0129777e-05;1.8332459e-05;1.8846954e-05;1.9476705e-05;2.0490046e-05;2.4588055e-05;3.1702259e-05;3.2989096e-05;3.4350234e-05;3.6132309e-05;4.3358771e-05;5.1589831e-05;5.3089863e-05;5.5504495e-05;5.7558217e-05;6.906986e-05;8.8425554e-05;9.0996626e-05;9.5135332e-05;9.8655434e-05;0.000118386521;0.000127762888;0.000131477737;0.000137457604;0.000142543673;0.000171052407;0.000173370104;0.000178411033;0.000186525519;0.00019342715;0.000232112579;0;0;0;0;0;2.7034922e-05;2.7736404e-05;2.8327181e-05;2.8334748e-05;3.4001697e-05;2.6405907e-05;2.7071047e-05;2.7741775e-05;2.8341663e-05;3.4009995e-05;2.8222037e-05;2.901408e-05;2.9983555e-05;3.154355e-05;3.785226e-05;4.6178646e-05;4.8053099e-05;5.0035781e-05;5.2631616e-05;6.3157939e-05;7.2338984e-05;7.444232e-05;7.7828104e-05;8.0707822e-05;9.6849386e-05;0.000103764515;0.000106781584;0.000111638221;0.000115768947;0.000138922737;0.000172183844;0.000177190281;0.000185249245;0.000192103652;0.000230524383;0.000226354181;0.000232935681;0.000243530056;0.000252540911;0.000303049093],[5 9 4]) % Wolfspeed XML derived J  Tj_loss=[25 75 125 150 900] % Wolfspeed XML derived degC  Iout_data_loss=[0 4.08 8.4 12.48 16.32 20.4 24.24 27.84 31.68] % Wolfspeed XML derived A  Vds_loss=[-10 0 600 800] % Wolfspeed XML derived V  Eon_scalar=22.86e-3 % Parameter not set J  Eoff_scalar=17.14e-3 % Parameter not set J  Voff=300 % Parameter not set V  Iout_scalar=600 % Parameter not set A  useCurrentFromPreviousCycle=false  useVoltageFromPreviousCycle=false  diodeModelType=ee.enum.converters.diodeModelType.tabulated  diodeTableType=ee.enum.diode.tableType.VfMat  diode_ReverseIVType=ee.enum.diode.diodeReverseIV.constant  diode_IfMat=[.07, .12, .19, 1.75, 4.24, 7.32, 11.2; .16, .3, .72, 2.14, 4.02, 6.35, 9.12] % Parameter not set A  diode_VfMat=[0 3.27 3.6 3.85 4.4 4.95 5.7 6.25 7 7.62;0 2.8 3.16 3.4 3.8 4.25 4.85 5.3 6 6.6;0 2.52 2.76 2.97 3.36 3.78 4.35 4.8 5.5 6.1;0 2.016 2.208 2.376 2.688 3.024 3.48 3.84 4.4 4.88] % Wolfspeed XML derived V  diode_TjVec=[-55 25 150 900] % Wolfspeed XML derived degC  diode_VfVec=[.5, .7, .9, 1.3, 1.7, 2.1, 2.5] % Parameter not set V  diode_IfVec=[0 0.3 1 2 5 10 20 30 50 70] % Wolfspeed XML derived A  diode_IrMat=[1e-06, 2e-06, 5e-06, 1e-05, 2.5e-05, 5e-05, .0001; 2e-06, 5e-06, 1e-05, 4e-05, 8e-05, .0002, .0005] % Parameter not set A  diode_VrMat=[10, 100, 200, 250, 300, 325, 350; 10, 70, 160, 220, 270, 300, 320] % Parameter not set V  diode_VrVec=[10, 20, 40, 50, 70, 80, 100] % Parameter not set V  diode_IrVec=[1e-06, 2e-06, 5e-06, 1e-05, 2e-05, 5e-05, .0001] % Parameter not set A  diode_Vr=-600 % Parameter not set V  diode_Ls=150 % Parameter not set nH  diode_Erec=0.03 % Parameter not set J  diode_rec_loss_model=ee.enum.diode.reverseRecoveryModelTabulateUpTo3D.fixed  diode_ErecVal=0 % Parameter not set J  diode_scaleWithIandV=false  diode_ErecMat=[0 0;0 0] % Wolfspeed XML derived J  diodeErecMat3D=zeros(2, 3, 2) % Parameter not set J  diode_TjrecVec=[25 35] % Wolfspeed XML derived degC  diode_IfrecVec=[0 10] % Wolfspeed XML derived A  diodeVrecVec=[0, 100] % Parameter not set V  diode_IrecVal=10 % Parameter not set A  diode_VrecVal=10 % Wolfspeed XML derived V  diode_tFilter=1 / 1000 / 100 % Parameter not set s  separateThermalPortForDiode=false  thermal_network_parameterization=ee.enum.thermalNetworkTopology.external  Rth=[.03, .2] % Parameter not set K/W  Rth_Cauer=[0.00956 0.242 0.167 0.228] % Wolfspeed XML derived K/W  Rth_Foster=[.08, .14, .22, .16] % Parameter not set K/W  thermal_mass_parameterization=ee.enum.thermalNetwork.thermalmass  thermal_mass=[3, 25] % Parameter not set J/K  thermal_mass_Cauer=[0.00156 0.00604 0.0619 0.358] % Wolfspeed XML derived J/K  thermal_mass_Foster=[.001, .005, .05, .5] % Parameter not set J/K  thermal_time_constant=[.1, 5] % Parameter not set s  thermal_time_constant_Cauer=[.1, 1, 5] % Parameter not set s  thermal_time_constant_Foster=[7e-05, .0007, .01, .08] % Parameter not set s  thermal_mass_initial_temperatures=[25, 25] % Parameter not set degC  thermal_mass_initial_temperatures_Cauer=[25 25 25 25] % Wolfspeed XML derived degC  junction_thermal_mass=0.1 % Parameter not set J/K  Tvec_initial_Foster=[25, 25, 25, 25] % Parameter not set degC  RthDiode=[.03, .2] % Parameter not set K/W  RthCauerDiode=[0.00956 0.242 0.167 0.228] % Wolfspeed XML derived K/W  RthFosterDiode=[.03, .2] % Parameter not set K/W  thermalMassDiode=[3, 25] % Parameter not set J/K  thermalMassCauerDiode=[0.00156 0.00604 0.0619 0.358] % Wolfspeed XML derived J/K  thermalMassFosterDiode=[33, 50] % Parameter not set J/K  thermalTauDiode=[.1, 5] % Parameter not set s  thermalTauCauerDiode=[.1, 1, 5] % Parameter not set s  thermalTauFosterDiode=[1, 10] % Parameter not set s  thermalMassInitTempDiode=[25, 25] % Parameter not set degC  thermalMassInitTempCauerDiode=[25 25 25 25] % Wolfspeed XML derived degC  junctionthermalMassDiode=0.1 % Parameter not set J/K  TVecInitialFosterDiode=[25, 25, 25, 25] % Parameter not set degC  no_thermal_network=0 % Parameter not set  mosfet_junction_temperature_specify=on  mosfet_junction_temperature_priority=High  mosfet_junction_temperature=simTempPri_K K  mosfet_junction_temperature_nominal_specify=off  mosfet_junction_temperature_nominal_value=1  mosfet_junction_temperature_nominal_unit=degC  diode_junction_temperature_specify=off  diode_junction_temperature_priority=None  diode_junction_temperature=simTempPri_K K  diode_junction_temperature_nominal_specify=off  diode_junction_temperature_nominal_value=1  diode_junction_temperature_nominal_unit=degC  Qj_specify=off  Qj_priority=None  Qj=0 W  Qj_nominal_specify=off  Qj_nominal_value=1  Qj_nominal_unit=W  accumulatedSwitchingLosses_specify=off  accumulatedSwitchingLosses_priority=None  accumulatedSwitchingLosses=0 J
      settings: AttributesFormatString=Wolfspeed:C2M0080120D
  PS-Simulink Converter1 : nesl_utility/PS-Simulink Converter  PhysicalDomain=network_engine_domain  SubClassName=ps_output  LeftPortType=input  RightPortType=output  PseudoPeriodic=off  Frequencies=[]  VectorFormat=inherit  Unit=inherit  AffineConversion=off
  SL_PS{1..4} (4 alike) : nesl_utility/Simulink-PS Converter  PhysicalDomain=network_engine_domain  SubClassName=ps_input  LeftPortType=input  RightPortType=output  PseudoPeriodic=off  Frequencies=[]  NoiseDistribution=none  NoiseParameters=[]  Unit=1  AffineConversion=off  FilteringAndDerivatives=provide  SimscapeFilterOrder=1  InputFilterTimeConstant=0.001  UdotUserProvided=0
  Temperature Source : fl_lib/Thermal/Thermal Sources/Temperature Source  temperature=simTempPri_K K
  Thermal Resistor{1..4} (4 alike) : ee_lib/Passive/Thermal/Thermal Resistor  R=1e-3 K/W  T_specify=on  T_priority=None  T=0 K  T_nominal_specify=off  T_nominal_value=1  T_nominal_unit=K  Q_specify=off  Q_priority=None  Q=0 W  Q_nominal_specify=off  Q_nominal_value=1  Q_nominal_unit=W
  VinP : PMIOPort  Side=Left
  VinN : PMIOPort  Port=2  Side=Left
  MidA : PMIOPort  Port=3  Side=Right
  MidB : PMIOPort  Port=4  Side=Right
  wires:
  G/1 -> Demux/1
  Demux/1 -> [G1]
  Demux/2 -> [G2]
  Demux/3 -> [G3]
  Demux/4 -> [G4]
  [G1] -> SL_PS1/1
  [G2] -> SL_PS2/1
  [G3] -> SL_PS3/1
  [G4] -> SL_PS4/1
  connections:
  MOSFETPriA2/LConn2 -- Thermal Resistor2/RConn1
  MOSFETPriA1/LConn2 -- Thermal Resistor1/RConn1
  SL_PS4/RConn1 -- MOSFETPriB2/LConn1
  SL_PS3/RConn1 -- MOSFETPriB1/LConn1
  SL_PS2/RConn1 -- MOSFETPriA2/LConn1
  SL_PS1/RConn1 -- MOSFETPriA1/LConn1
  Thermal Resistor1/LConn1 -- Thermal Resistor3/LConn1 -- Thermal Resistor4/LConn1 -- Thermal Resistor2/LConn1 -- Temperature Source/LConn1
  Thermal Resistor3/RConn1 -- MOSFETPriB1/LConn2
  Thermal Resistor4/RConn1 -- MOSFETPriB2/LConn2
  MOSFETPriA1/RConn2 -- Cds1/RConn1 -- Cds2/LConn1 -- MOSFETPriA2/RConn1 -- MidA/RConn1
  MOSFETPriA1/RConn1 -- Cds3/LConn1 -- MOSFETPriB1/RConn1 -- VinP/RConn1 -- Cds1/LConn1
  MOSFETPriB1/RConn2 -- Cds3/RConn1 -- MidB/RConn1 -- Cds4/LConn1 -- MOSFETPriB2/RConn1
  MOSFETPriB2/RConn2 -- Cds4/RConn1 -- VinN/RConn1 -- MOSFETPriA2/RConn2 -- Cds2/RConn1
